simulink model "arducopter"  (R2024b)
settings: Solver=FixedStepAuto  StartTime=0.0  StopTime=simIn.param.timeEnd  FixedStep=simIn.param.dt  RelTol=1e-3
undefined symbols (not defined in the file or in its folder): DiscIntNeverNeededParam, sim, simIn
libraries: simulink x60, slident x4, vrlib x1
(part 4 of 9)

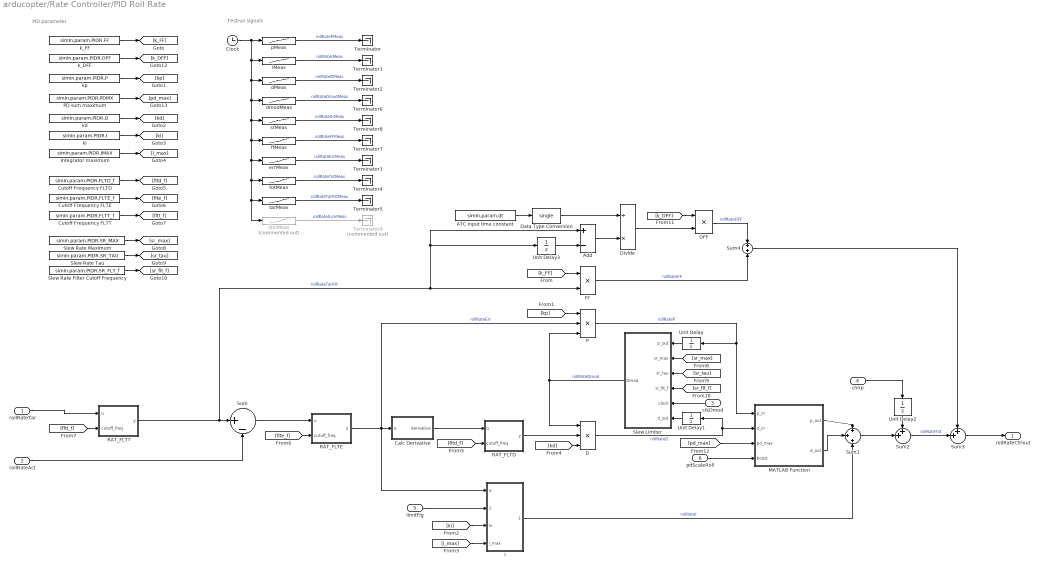
== system arducopter/Rate Controller/PID Roll Rate ==
  note: Testrun signals
  note: PID parameter
  rollRateTar : Inport
  rollRateAct : Inport  Port=2
  clkDmod : Inport  Port=3
  chirp : Inport  Port=4
  limitFlg : Inport  Port=5
  pdScaleRoll : Inport  Port=6
  ATC input time constant : Constant  Value=simIn.param.dt
  Add : Sum  Inputs=+-
  Calc Derivative : Subsystem
  Clock : Clock
  Cutoff Frequency FLTD : Constant  Value=simIn.param.PIDR.FLTD_f
  Cutoff Frequency FLTE : Constant  Value=simIn.param.PIDR.FLTE_f
  Cutoff Frequency FLTT : Constant  Value=simIn.param.PIDR.FLTT_f
  D : Product  Inputs=3
  DFF : Product
  Data Type Conversion : DataTypeConversion  OutDataTypeStr=single  SaturateOnIntegerOverflow=off  RndMeth=Floor
  Divide : Product  Inputs=/*
  FF : Product
  I : Subsystem
  Integrator maximum : Constant  Value=simIn.param.PIDR.IMAX
  MATLAB Function : MATLAB Function  TreatAsAtomicUnit=on
  P : Product  Inputs=3
  PD sum maximum : Constant  Value=simIn.param.PIDR.PDMX
  RAT_FLTD : Subsystem  TreatAsAtomicUnit=on  SystemSampleTime=simIn.param.dt
  RAT_FLTE : Subsystem  TreatAsAtomicUnit=on  SystemSampleTime=simIn.param.dt
  RAT_FLTT : Subsystem  TreatAsAtomicUnit=on  SystemSampleTime=simIn.param.dt
  Slew Limiter : Subsystem
  Slew Rate Filter Cutoff Frequency : Constant  Value=simIn.param.PIDR.SR_FLT_f
  Slew Rate Maximum : Constant  Value=simIn.param.PIDR.SR_MAX
  Slew Rate Tau : Constant  Value=simIn.param.PIDR.SR_TAU
  Sum : Sum  Inputs=|+-
  Sum1 : Sum  Inputs=+|+|+
  Sum2 : Sum  Inputs=++|
  Sum3 : Sum  Inputs=++|  OutDataTypeStr=single
  Sum4 : Sum
  Terminator{,1..8} (9 alike) : Terminator
  Terminator9 : Terminator  Commented=on
  Unit Delay : UnitDelay  InitialCondition=simIn.init.PIDR.P  SampleTime=-1  HasFrameUpgradeWarning=on
  Unit Delay1 : UnitDelay  InitialCondition=simIn.init.PIDR.D  SampleTime=-1  HasFrameUpgradeWarning=on
  Unit Delay2 : UnitDelay  SampleTime=-1  HasFrameUpgradeWarning=on
  Unit Delay3 : UnitDelay  SampleTime=-1  HasFrameUpgradeWarning=on
  dMeas : Lookup_n-D  NumberOfTableDimensions=1  BreakpointsForDimension1=simIn.signals.PIDR.Time  Table=simIn.signals.PIDR.D  InternalRulePriority=Speed  RndMeth=Simplest
  dmodMeas : Lookup_n-D  NumberOfTableDimensions=1  BreakpointsForDimension1=simIn.signals.PIDR.Time  Table=simIn.signals.PIDR.DMod  InternalRulePriority=Speed  RndMeth=Simplest
  errMeas : Lookup_n-D  NumberOfTableDimensions=1  BreakpointsForDimension1=simIn.signals.PIDR.Time  Table=simIn.signals.PIDR.Err  InternalRulePriority=Speed  RndMeth=Simplest
  ffMeas : Lookup_n-D  NumberOfTableDimensions=1  BreakpointsForDimension1=simIn.signals.PIDR.Time  Table=simIn.signals.PIDR.FF  InternalRulePriority=Speed  RndMeth=Simplest
  iMeas : Lookup_n-D  NumberOfTableDimensions=1  BreakpointsForDimension1=simIn.signals.PIDR.Time  Table=simIn.signals.PIDR.I  InternalRulePriority=Speed  RndMeth=Simplest
  ilimMeas : Lookup_n-D  Commented=on  NumberOfTableDimensions=1  BreakpointsForDimension1=simIn.signals.PIDR.Time  Table=simIn.signals.PIDR.ILimit  InternalRulePriority=Speed  RndMeth=Simplest
  k_DFF : Constant  Value=simIn.param.PIDR.DFF
  k_FF : Constant  Value=simIn.param.PIDR.FF
  kd : Constant  Value=simIn.param.PIDR.D
  ki : Constant  Value=simIn.param.PIDR.I
  kp : Constant  Value=simIn.param.PIDR.P
  pMeas : Lookup_n-D  NumberOfTableDimensions=1  BreakpointsForDimension1=simIn.signals.PIDR.Time  Table=simIn.signals.PIDR.P  InternalRulePriority=Speed  RndMeth=Simplest
  srMeas : Lookup_n-D  NumberOfTableDimensions=1  BreakpointsForDimension1=simIn.signals.PIDR.Time  Table=simIn.signals.PIDR.SRate  InternalRulePriority=Speed  RndMeth=Simplest
  tarMeas : Lookup_n-D  NumberOfTableDimensions=1  BreakpointsForDimension1=simIn.signals.PIDR.Time  Table=simIn.signals.PIDR.Tar  InternalRulePriority=Speed  RndMeth=Simplest
  totMeas : Lookup_n-D  NumberOfTableDimensions=1  BreakpointsForDimension1=simIn.signals.RATE.Time  Table=simIn.signals.RATE.ROut  InternalRulePriority=Speed  RndMeth=Simplest
  rollRateCtrlout : Outport
  wires:
  RAT_FLTD/1(y) -> D/2
  RAT_FLTE/1(y) -> P/2, Calc Derivative/1(e), I/1(e)  "rollRateErr"
  limitFlg/1 -> I/2(limit_flg)
  P/1 -> MATLAB Function/1(p_in), Unit Delay/1  "rollRateP"
  D/1 -> Unit Delay1/1, MATLAB Function/2(d_in)  "rollRateD"
  I/1(integrator) -> Sum1/3  "rollRateI"
  Sum3/1 -> rollRateCtrlout/1
  RAT_FLTT/1(y) -> Add/1, Unit Delay3/1, FF/2, Sum/1  "rollRateTarFilt"
  rollRateTar/1 -> RAT_FLTT/1(u)
  rollRateAct/1 -> Sum/2
  Sum/1 -> RAT_FLTE/1(u)
  k_FF/1 -> [k_FF]
  kp/1 -> [kp]
  kd/1 -> [kd]
  ki/1 -> [ki]
  Integrator maximum/1 -> [i_max]
  Cutoff Frequency FLTD/1 -> [fltd_f]
  Cutoff Frequency FLTE/1 -> [flte_f]
  Cutoff Frequency FLTT/1 -> [fltt_f]
  [k_FF] -> FF/1
  [kp] -> P/1
  [ki] -> I/3(ki)
  [i_max] -> I/4(i_max)
  [kd] -> D/3
  [fltd_f] -> RAT_FLTD/2(cutoff_freq)
  [flte_f] -> RAT_FLTE/2(cutoff_freq)
  [fltt_f] -> RAT_FLTT/2(cutoff_freq)
  Sum2/1 -> Sum3/2  "rollRateTot"
  pMeas/1 -> Terminator/1  "rollRatePMeas"
  iMeas/1 -> Terminator1/1  "rollRateIMeas"
  errMeas/1 -> Terminator3/1  "rollRateErrMeas"
  dMeas/1 -> Terminator2/1  "rollRateDMeas"
  tarMeas/1 -> Terminator5/1  "rollRateTarFiltMeas"
  totMeas/1 -> Terminator4/1  "rollRateTotMeas"
  Unit Delay/1 -> Slew Limiter/1(p_out)
  Unit Delay1/1 -> Slew Limiter/6(d_out)
  Slew Rate Maximum/1 -> [sr_max]
  [sr_max] -> Slew Limiter/2(sr_max)
  Slew Rate Tau/1 -> [sr_tau]
  Slew Rate Filter Cutoff Frequency/1 -> [sr_flt_f]
  [sr_tau] -> Slew Limiter/3(sr_tau)
  [sr_flt_f] -> Slew Limiter/4(sr_flt_f)
  Slew Limiter/1(Dmod) -> P/3, D/1  "rollRateDmod"
  Sum1/1 -> Sum2/2
  chirp/1 -> Unit Delay2/1
  Unit Delay2/1 -> Sum2/1
  Calc Derivative/1(derivative) -> RAT_FLTD/1(u)
  dmodMeas/1 -> Terminator6/1  "rollRateDmodMeas"
  ffMeas/1 -> Terminator7/1  "rollRateFFMeas"
  srMeas/1 -> Terminator8/1  "rollRateSrMeas"
  clkDmod/1 -> Slew Limiter/5(clock)
  ilimMeas/1 -> Terminator9/1  "rollRateILimMeas"
  Clock/1 -> ilimMeas/1, tarMeas/1, totMeas/1, errMeas/1, ffMeas/1, srMeas/1, dmodMeas/1, dMeas/1, iMeas/1, pMeas/1
  FF/1 -> Sum4/2  "rollRateFF"
  k_DFF/1 -> [k_DFF]
  Unit Delay3/1 -> Add/2
  [k_DFF] -> DFF/1
  DFF/1 -> Sum4/1  "rollRateDFF"
  Sum4/1 -> Sum3/1
  PD sum maximum/1 -> [pd_max]
  Data Type Conversion/1 -> Divide/1
  ATC input time constant/1 -> Data Type Conversion/1
  Add/1 -> Divide/2
  Divide/1 -> DFF/2
  MATLAB Function/2(d_out) -> Sum1/2
  MATLAB Function/1(p_out) -> Sum1/1
  [pd_max] -> MATLAB Function/3(pd_max)
  pdScaleRoll/1 -> MATLAB Function/4(boost)

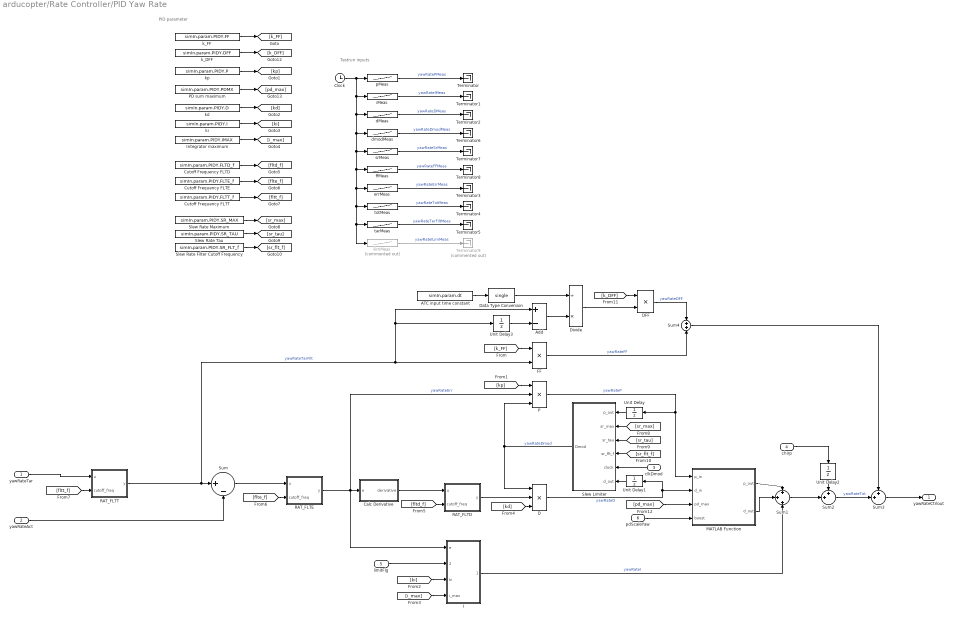
== system arducopter/Rate Controller/PID Yaw Rate ==
  note: Testrun inputs
  note: PID parameter
  yawRateTar : Inport
  yawRateAct : Inport  Port=2
  clkDmod : Inport  Port=3
  chirp : Inport  Port=4
  limitFlg : Inport  Port=5
  pdScaleYaw : Inport  Port=6
  ATC input time constant : Constant  Value=simIn.param.dt
  Add : Sum  Inputs=+-
  Calc Derivative : Subsystem
  Clock : Clock
  Cutoff Frequency FLTD : Constant  Value=simIn.param.PIDY.FLTD_f
  Cutoff Frequency FLTE : Constant  Value=simIn.param.PIDY.FLTE_f
  Cutoff Frequency FLTT : Constant  Value=simIn.param.PIDY.FLTT_f
  D : Product  Inputs=3
  DFF : Product
  Data Type Conversion : DataTypeConversion  OutDataTypeStr=single  SaturateOnIntegerOverflow=off  RndMeth=Floor
  Divide : Product  Inputs=/*
  FF : Product
  I : Subsystem
  Integrator maximum : Constant  Value=simIn.param.PIDY.IMAX
  MATLAB Function : MATLAB Function  TreatAsAtomicUnit=on
  P : Product  Inputs=3
  PD sum maximum : Constant  Value=simIn.param.PIDY.PDMX
  RAT_FLTD : Subsystem  TreatAsAtomicUnit=on  SystemSampleTime=simIn.param.dt
  RAT_FLTE : Subsystem  TreatAsAtomicUnit=on  SystemSampleTime=simIn.param.dt
  RAT_FLTT : Subsystem  TreatAsAtomicUnit=on  SystemSampleTime=simIn.param.dt
  Slew Limiter : Subsystem
  Slew Rate Filter Cutoff Frequency : Constant  Value=simIn.param.PIDY.SR_FLT_f
  Slew Rate Maximum : Constant  Value=simIn.param.PIDY.SR_MAX
  Slew Rate Tau : Constant  Value=simIn.param.PIDY.SR_TAU
  Sum : Sum  Inputs=|+-
  Sum1 : Sum  Inputs=+|+|+
  Sum2 : Sum  Inputs=++|
  Sum3 : Sum  Inputs=++|  OutDataTypeStr=single
  Sum4 : Sum
  Terminator{,1..8} (9 alike) : Terminator
  Terminator9 : Terminator  Commented=on
  Unit Delay : UnitDelay  InitialCondition=simIn.init.PIDY.P  SampleTime=-1  HasFrameUpgradeWarning=on
  Unit Delay1 : UnitDelay  InitialCondition=simIn.init.PIDY.D  SampleTime=-1  HasFrameUpgradeWarning=on
  Unit Delay2 : UnitDelay  SampleTime=-1  HasFrameUpgradeWarning=on
  Unit Delay3 : UnitDelay  SampleTime=-1  HasFrameUpgradeWarning=on
  dMeas : Lookup_n-D  NumberOfTableDimensions=1  BreakpointsForDimension1=simIn.signals.PIDY.Time  Table=simIn.signals.PIDY.D  InternalRulePriority=Speed  RndMeth=Simplest
  dmodMeas : Lookup_n-D  NumberOfTableDimensions=1  BreakpointsForDimension1=simIn.signals.PIDY.Time  Table=simIn.signals.PIDY.DMod  InternalRulePriority=Speed  RndMeth=Simplest
  errMeas : Lookup_n-D  NumberOfTableDimensions=1  BreakpointsForDimension1=simIn.signals.PIDY.Time  Table=simIn.signals.PIDY.Err  InternalRulePriority=Speed  RndMeth=Simplest
  ffMeas : Lookup_n-D  NumberOfTableDimensions=1  BreakpointsForDimension1=simIn.signals.PIDY.Time  Table=simIn.signals.PIDY.FF  InternalRulePriority=Speed  RndMeth=Simplest
  iMeas : Lookup_n-D  NumberOfTableDimensions=1  BreakpointsForDimension1=simIn.signals.PIDY.Time  Table=simIn.signals.PIDY.I  InternalRulePriority=Speed  RndMeth=Simplest
  ilimMeas : Lookup_n-D  Commented=on  NumberOfTableDimensions=1  BreakpointsForDimension1=simIn.signals.PIDY.Time  Table=simIn.signals.PIDY.ILimit  InternalRulePriority=Speed  RndMeth=Simplest
  k_DFF : Constant  Value=simIn.param.PIDY.DFF
  k_FF : Constant  Value=simIn.param.PIDY.FF
  kd : Constant  Value=simIn.param.PIDY.D
  ki : Constant  Value=simIn.param.PIDY.I
  kp : Constant  Value=simIn.param.PIDY.P
  pMeas : Lookup_n-D  NumberOfTableDimensions=1  BreakpointsForDimension1=simIn.signals.PIDY.Time  Table=simIn.signals.PIDY.P  InternalRulePriority=Speed  RndMeth=Simplest
  srMeas : Lookup_n-D  NumberOfTableDimensions=1  BreakpointsForDimension1=simIn.signals.PIDY.Time  Table=simIn.signals.PIDY.SRate  InternalRulePriority=Speed  RndMeth=Simplest
  tarMeas : Lookup_n-D  NumberOfTableDimensions=1  BreakpointsForDimension1=simIn.signals.PIDY.Time  Table=simIn.signals.PIDY.Tar  InternalRulePriority=Speed  RndMeth=Simplest
  totMeas : Lookup_n-D  NumberOfTableDimensions=1  BreakpointsForDimension1=simIn.signals.RATE.Time  Table=simIn.signals.RATE.YOut  InternalRulePriority=Speed  RndMeth=Simplest
  yawRateCtrlout : Outport
  wires:
  pMeas/1 -> Terminator/1  "yawRatePMeas"
  iMeas/1 -> Terminator1/1  "yawRateIMeas"
  dMeas/1 -> Terminator2/1  "yawRateDMeas"
  totMeas/1 -> Terminator4/1  "yawRateTotMeas"
  tarMeas/1 -> Terminator5/1  "yawRateTarFiltMeas"
  errMeas/1 -> Terminator3/1  "yawRateErrMeas"
  dmodMeas/1 -> Terminator6/1  "yawRateDmodMeas"
  srMeas/1 -> Terminator7/1  "yawRateSrMeas"
  ffMeas/1 -> Terminator8/1  "yawRateFFMeas"
  ilimMeas/1 -> Terminator9/1  "yawRateILimMeas"
  Clock/1 -> ilimMeas/1, tarMeas/1, totMeas/1, errMeas/1, ffMeas/1, srMeas/1, dmodMeas/1, dMeas/1, iMeas/1, pMeas/1
  Sum/1 -> RAT_FLTE/1(u)
  Slew Limiter/1(Dmod) -> P/3, D/1  "yawRateDmod"
  P/1 -> MATLAB Function/1(p_in), Unit Delay/1  "yawRateP"
  [fltt_f] -> RAT_FLTT/2(cutoff_freq)
  Unit Delay/1 -> Slew Limiter/1(p_out)
  FF/1 -> Sum4/2  "yawRateFF"
  DFF/1 -> Sum4/1  "yawRateDFF"
  MATLAB Function/2(d_out) -> Sum1/2
  MATLAB Function/1(p_out) -> Sum1/1
  [i_max] -> I/4(i_max)
  Calc Derivative/1(derivative) -> RAT_FLTD/1(u)
  I/1(integrator) -> Sum1/3  "yawRateI"
  Unit Delay2/1 -> Sum2/1
  [sr_tau] -> Slew Limiter/3(sr_tau)
  [flte_f] -> RAT_FLTE/2(cutoff_freq)
  [sr_flt_f] -> Slew Limiter/4(sr_flt_f)
  [pd_max] -> MATLAB Function/3(pd_max)
  Unit Delay1/1 -> Slew Limiter/6(d_out)
  [kp] -> P/1
  yawRateTar/1 -> RAT_FLTT/1(u)
  chirp/1 -> Unit Delay2/1
  D/1 -> Unit Delay1/1, MATLAB Function/2(d_in)  "yawRateD"
  RAT_FLTD/1(y) -> D/2
  [k_FF] -> FF/1
  ATC input time constant/1 -> Data Type Conversion/1
  Data Type Conversion/1 -> Divide/1
  [ki] -> I/3(ki)
  Sum3/1 -> yawRateCtrlout/1
  Add/1 -> Divide/2
  RAT_FLTE/1(y) -> P/2, Calc Derivative/1(e), I/1(e)  "yawRateErr"
  limitFlg/1 -> I/2(limit_flg)
  clkDmod/1 -> Slew Limiter/5(clock)
  [fltd_f] -> RAT_FLTD/2(cutoff_freq)
  Sum4/1 -> Sum3/1
  [k_DFF] -> DFF/1
  Sum1/1 -> Sum2/2
  [sr_max] -> Slew Limiter/2(sr_max)
  Divide/1 -> DFF/2
  [kd] -> D/3
  RAT_FLTT/1(y) -> Add/1, Unit Delay3/1, FF/2, Sum/1  "yawRateTarFilt"
  Unit Delay3/1 -> Add/2
  Sum2/1 -> Sum3/2  "yawRateTot"
  yawRateAct/1 -> Sum/2
  Integrator maximum/1 -> [i_max]
  Slew Rate Maximum/1 -> [sr_max]
  ki/1 -> [ki]
  Cutoff Frequency FLTD/1 -> [fltd_f]
  Cutoff Frequency FLTE/1 -> [flte_f]
  k_FF/1 -> [k_FF]
  Slew Rate Tau/1 -> [sr_tau]
  PD sum maximum/1 -> [pd_max]
  k_DFF/1 -> [k_DFF]
  Slew Rate Filter Cutoff Frequency/1 -> [sr_flt_f]
  kp/1 -> [kp]
  Cutoff Frequency FLTT/1 -> [fltt_f]
  kd/1 -> [kd]
  pdScaleYaw/1 -> MATLAB Function/4(boost)

== system arducopter/Throttle/Input Handler ==
  note: Input Handler
      | Determines source of the inputs to the subsystem, which can
      | be either the real flight data or simulated data.
  inMeas : Inport
  inSim : Inport  Port=2
  thrMan : Inport  Port=3
  Bus Creator : BusCreator  Inputs=9
  Bus Selector : BusSelector  OutputSignals=throttle.thrIn
  Bus Selector1 : BusSelector  OutputSignals=CTUN.thrInMeas,CTUN.angBst,BAT.batRestVoltEst,BAT.batCurr,BAT.batRes,BAT.batVolt,BARO.baroAlt,BARO.baroAirPress,BARO.baroGndTemp
  Switch : Switch  Criteria=u2 > Threshold  SaturateOnIntegerOverflow=off  InputSameDT=off
  data_in : Outport
  wires:
  inSim/1 -> Bus Selector/1
  inMeas/1 -> Bus Selector1/1
  thrMan/1 -> Switch/2
  Bus Selector/1 -> Switch/3  "<thrIn>"
  Bus Selector1/1 -> Switch/1  "<thrInMeas>"
  Bus Selector1/9 -> Bus Creator/9  "<baroGndTemp>"
  Bus Selector1/8 -> Bus Creator/8  "<baroAirPress>"
  Bus Selector1/7 -> Bus Creator/7  "<baroAlt>"
  Bus Selector1/6 -> Bus Creator/6  "<batVolt>"
  Bus Selector1/5 -> Bus Creator/5  "<batRes>"
  Bus Selector1/4 -> Bus Creator/4  "<batCurr>"
  Bus Selector1/3 -> Bus Creator/3  "<batRestVoltEst>"
  Bus Selector1/2 -> Bus Creator/2  "<angBst>"
  Switch/1 -> Bus Creator/1  "thrTar"
  Bus Creator/1 -> data_in/1

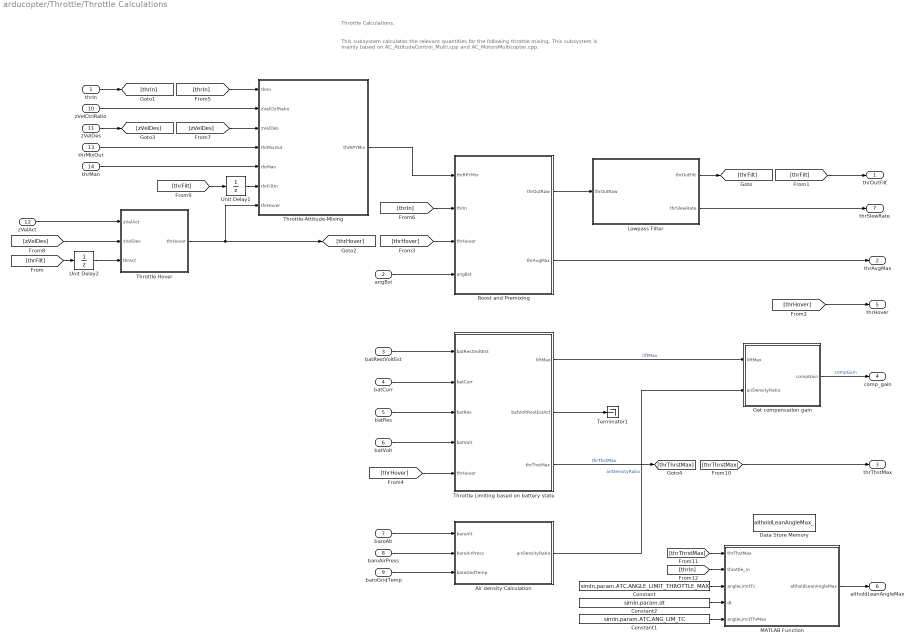
== system arducopter/Throttle/Throttle Calculations ==
  note: Throttle Calculations.
  note: This subsystem calculates the relevant quantities for the following throttle mixing.
      | This subsystem is mainly based on AC_AttitudeControl_Multi.cpp and AC_MotorsMulticopter.cpp.
  thrIn : Inport
  angBst : Inport  Port=2
  batRestVoltEst : Inport  Port=3
  batCurr : Inport  Port=4
  batRes : Inport  Port=5
  batVolt : Inport  Port=6
  baroAlt : Inport  Port=7
  baroAirPress : Inport  Port=8
  baroGndTemp : Inport  Port=9
  zVelCtrlRatio : Inport  Port=10
  zVelDes : Inport  Port=11
  zVelAct : Inport  Port=12
  thrMixOut : Inport  Port=13
  thrMan : Inport  Port=14
  Air density Calculation : Subsystem
  Boost and Premixing : Subsystem  TreatAsAtomicUnit=on  SystemSampleTime=simIn.param.dt
  Constant : Constant  Value=simIn.param.ATC.ANGLE_LIMIT_THROTTLE_MAX
  Constant1 : Constant  Value=simIn.param.ATC.ANG_LIM_TC
  Constant2 : Constant  Value=simIn.param.dt
  Data Store Memory : DataStoreMemory  DataStoreName=altholdLeanAngleMax_  ReadBeforeWriteMsg=warning  WriteAfterWriteMsg=warning  WriteAfterReadMsg=warning  InitialValue=single(0)  ShowAdditionalParam=off  OutDataTypeStr=single
  Get compensation gain : MATLAB Function  TreatAsAtomicUnit=on
  Lowpass Filter : Subsystem
  MATLAB Function : MATLAB Function  TreatAsAtomicUnit=on
  Terminator1 : Terminator
  Throttle Hover : Subsystem  TreatAsAtomicUnit=on  SystemSampleTime=0.1
  Throttle Limiting based on battery state : Subsystem
  Throttle-Attitude-Mixing : Subsystem
  Unit Delay1 : UnitDelay  InitialCondition=simIn.init.CTUN.ThrOut  SampleTime=-1  HasFrameUpgradeWarning=on
  Unit Delay2 : UnitDelay  InitialCondition=simIn.init.CTUN.ThrOut  SampleTime=-1  HasFrameUpgradeWarning=on
  thrOutFilt : Outport
  thrAvgMax : Outport  Port=2
  thrThstMax : Outport  Port=3
  comp_gain : Outport  Port=4
  thrHover : Outport  Port=5
  altholdLeanAngleMax : Outport  Port=6
  thrSlewRate : Outport  Port=7
  wires:
  Throttle Hover/1(thrHover) -> [thrHover], Throttle-Attitude-Mixing/7(thrHover)
  Get compensation gain/1(compGain) -> comp_gain/1  "compGain"
  Throttle Limiting based on battery state/1(liftMax) -> Get compensation gain/1(liftMax)  "liftMax"
  [thrFilt] -> Unit Delay2/1
  Throttle Limiting based on battery state/2(batVoltRestEstAct) -> Terminator1/1
  [thrHover] -> Throttle Limiting based on battery state/5(thrHover)
  Unit Delay2/1 -> Throttle Hover/3(thrAct)
  Throttle Limiting based on battery state/3(thrThstMax) -> [thrThrstMax]  "thrThstMax"
  [thrFilt] -> thrOutFilt/1
  Lowpass Filter/1(thrOutFilt) -> [thrFilt]
  angBst/1 -> Boost and Premixing/4(angBst)
  [thrHover] -> Boost and Premixing/3(thrHover)
  Boost and Premixing/2(thrAvgMax) -> thrAvgMax/1
  batRestVoltEst/1 -> Throttle Limiting based on battery state/1(batRestVoltEst)
  batCurr/1 -> Throttle Limiting based on battery state/2(batCurr)
  batRes/1 -> Throttle Limiting based on battery state/3(batRes)
  batVolt/1 -> Throttle Limiting based on battery state/4(batVolt)
  baroAlt/1 -> Air density Calculation/1(baroAlt)
  baroAirPress/1 -> Air density Calculation/2(baroAirPress)
  baroGndTemp/1 -> Air density Calculation/3(baroGndTemp)
  Boost and Premixing/1(thrOutRaw) -> Lowpass Filter/1(thrOutRaw)
  [thrHover] -> thrHover/1
  [thrIn] -> Boost and Premixing/2(thrIn)
  thrIn/1 -> [thrIn]
  zVelCtrlRatio/1 -> Throttle-Attitude-Mixing/2(zVelCtrlRatio)
  thrMan/1 -> Throttle-Attitude-Mixing/5(thrMan)
  Throttle-Attitude-Mixing/1(thrRPYMix) -> Boost and Premixing/1(thrRPYMix)
  [thrIn] -> Throttle-Attitude-Mixing/1(thrIn)
  zVelDes/1 -> [zVelDes]
  [zVelDes] -> Throttle-Attitude-Mixing/3(zVelDes)
  [zVelDes] -> Throttle Hover/2(zVelDes)
  zVelAct/1 -> Throttle Hover/1(zVelAct)
  Air density Calculation/1(airDensityRatio) -> Get compensation gain/2(airDensityRatio)  "airDensityRatio"
  thrMixOut/1 -> Throttle-Attitude-Mixing/4(thrMixOut)
  [thrFilt] -> Unit Delay1/1
  Unit Delay1/1 -> Throttle-Attitude-Mixing/6(thrFiltIn)
  [thrThrstMax] -> thrThstMax/1
  [thrThrstMax] -> MATLAB Function/1(thrThstMax)
  [thrIn] -> MATLAB Function/2(throttle_in)
  Constant/1 -> MATLAB Function/3(angleLimitTc)
  Constant1/1 -> MATLAB Function/5(angleLimitThrMax)
  Constant2/1 -> MATLAB Function/4(dt)
  MATLAB Function/1(altholdLeanAngleMax) -> altholdLeanAngleMax/1
  Lowpass Filter/2(thrSlewRate) -> thrSlewRate/1

== system arducopter/Attitude Controller/input_euler_angle_roll_pitch_euler_rate_yaw()/Add feedforward to angVelBody ==
  note: Thrust error angle above which yaw corrections are limited
  angVelBodyFeedforward : Inport
  angVelBodyIn : Inport  Port=2
  thurstErrorAngle : Inport  Port=3
  yawRateAct : Inport  Port=4
  Constant : Constant  Value=simIn.param.ATC.THRUST_ERROR_ANGLE
  MATLAB Function : MATLAB Function  TreatAsAtomicUnit=on
  angVelBody : Outport
  feedforwardScaler : Outport  Port=2
  wires:
  angVelBodyFeedforward/1 -> MATLAB Function/1(angVelBodyFeedforward)
  angVelBodyIn/1 -> MATLAB Function/2(angVelBodyIn)
  thurstErrorAngle/1 -> MATLAB Function/3(thrustErrorAngle)
  yawRateAct/1 -> MATLAB Function/4(yawRateAct)
  MATLAB Function/1(angVelBodyNew) -> angVelBody/1
  Constant/1 -> MATLAB Function/5(maxThrustErrorAngle4YawCorr)
  MATLAB Function/2(feedforwardScaler) -> feedforwardScaler/1

== system arducopter/Attitude Controller/input_euler_angle_roll_pitch_euler_rate_yaw()/Feedforward disabled ==
  note: QuaternionT<T>::from_euler()
      | Computes the quaternion from the given euler angles
  note: This subsystem represents to part of input_euler_angle_roll_pitch_euler_rate_yaw() that is executed, when the feedforward is disabled ( ATC_RATE_FF_ENAB = 0 )
  eulerAngleTar : Inport
  eulerInputDes : Inport  Port=2
  Constant : Constant  Value=0  OutDataTypeStr=single
  Constant1 : Constant  Value=0  OutDataTypeStr=single
  Demux : Demux  Outputs=3
  Gain : Gain  Gain=simIn.param.dt
  MATLAB Function : MATLAB Function  TreatAsAtomicUnit=on
  Selector : Selector  InputPortWidth=3  IndexOptions=Index vector (dialog)  Indices=[3]  OutputSizes=1
  Sum : Sum  Inputs=|++
  eulerRateTar : Outport
  angVelTar : Outport  Port=2
  attitudeTarget : Outport  Port=3
  wires:
  MATLAB Function/1(q) -> attitudeTarget/1  "attitudeTarget"
  Demux/1 -> MATLAB Function/1(roll)
  Demux/2 -> MATLAB Function/2(pitch)
  eulerInputDes/1 -> Demux/1
  Demux/3 -> Gain/1
  Gain/1 -> Sum/1
  Sum/1 -> MATLAB Function/3(yaw)
  eulerAngleTar/1 -> Selector/1
  Constant/1 -> eulerRateTar/1
  Constant1/1 -> angVelTar/1
  Selector/1 -> Sum/2

== system arducopter/Attitude Controller/input_euler_angle_roll_pitch_euler_rate_yaw()/Feedforward enabled ==
  note: direkt _attitude_target statt euler_angle_target
  note: euler_rate_to_ang_vel()
      | Converts the target euler rates into a target frame angular velocity vector for feedforward
  note: euler_accel_limit()
      | Translation of acceleration limits eulerAccelMax to the body frame
  note: This subsystem represents to part of input_euler_angle_roll_pitch_euler_rate_yaw() that is executed, when the feedforward is enabled (ATC_RATE_FF_ENAB = 1)
  note: Maximum angular accelerations in earth frame
  note: Input shaping
      | Computes target euler rates based on the error between latest angle target and the desired angle by the pilot, thereby considering acceleration limits.
  note: ang_vel_limit()
      | Ensures that angular velocites do not go over configured rate limits
  note: ang_vel_to_euler_rate()
      | Converts the target body-frame angular velocites into target euler rates
  eulerRateTarIn : Inport
  eulerAngleTar : Inport  Port=2
  eulerInputDes : Inport  Port=3
  Constant : Constant  Value=simIn.param.ATC.ACCEL_R_MAX
  Constant1 : Constant  Value=simIn.param.ATC.ACCEL_P_MAX
  Constant2 : Constant  Value=simIn.param.ATC.ACCEL_Y_MAX
  Constant3 : Constant  Value=simIn.param.ATC.RATE_R_MAX
  Constant4 : Constant  Value=simIn.param.ATC.RATE_P_MAX
  Constant5 : Constant  Value=simIn.param.ATC.RATE_Y_MAX
  Gain : Gain  Gain=pi/180
  Gain1 : Gain  Gain=pi/180
  Gain2 : Gain  Gain=pi/180
  MATLAB Function : MATLAB Function  TreatAsAtomicUnit=on
  MATLAB Function1 : MATLAB Function  TreatAsAtomicUnit=on
  MATLAB Function2 : MATLAB Function  TreatAsAtomicUnit=on
  MATLAB Function3 : MATLAB Function  TreatAsAtomicUnit=on
  Mux : Mux  Inputs=3
  cdeg/ss to rad/ss : Gain  Gain=0.01*pi/180
  input shaping : Subsystem
  eulerRateTarOut : Outport
  angVelTar : Outport  Port=2
  wires:
  [eulerAngleTar] -> MATLAB Function/1(eulerAngleTar), MATLAB Function1/1(eulerAngle), input shaping/1(eulerAngleTar)
  Constant/1 -> Mux/1
  Mux/1 -> cdeg/ss to rad/ss/1
  Constant1/1 -> Mux/2
  Constant2/1 -> Mux/3
  MATLAB Function/1(eulerAccelMaxBF) -> input shaping/4(eulerAccelMax)
  eulerInputDes/1 -> input shaping/2(eulerInputDes)
  eulerRateTarIn/1 -> input shaping/3(eulerRateTarIn)
  input shaping/1(eulerRateTar) -> MATLAB Function1/2(eulerRate)  "eulerRateTar"
  MATLAB Function1/1(angVelTar) -> MATLAB Function2/1(angVelTar)  "angVelTar"
  Gain/1 -> MATLAB Function2/2(angVelRollMax)
  Constant3/1 -> Gain/1
  Constant4/1 -> Gain1/1
  Gain1/1 -> MATLAB Function2/3(angVelPitchMax)
  Gain2/1 -> MATLAB Function2/4(angVelYawMax)
  Constant5/1 -> Gain2/1
  eulerAngleTar/1 -> [eulerAngleTar]  "eulerAngleTar"
  [eulerAngleTar] -> MATLAB Function3/2(eulerAngle)
  MATLAB Function3/1(eulerRate) -> eulerRateTarOut/1
  MATLAB Function2/1(angVelTarLimited) -> [angVelTar]
  [angVelTar] -> MATLAB Function3/1(angVelBf)
  [angVelTar] -> angVelTar/1
  cdeg/ss to rad/ss/1 -> MATLAB Function/2(eulerAccelMaxEF)

== system arducopter/Attitude Controller/input_euler_angle_roll_pitch_euler_rate_yaw()/Update attitudeTarget ==
  note: Normalize attitudeTarget
  note: Use angVelTar to rotate attitudeTarget
  note: Use rotated attitudeTarget, if FF is enabled.
      | Otherwise, use unchanged attitudeTarget
  attitudeTarget : Inport
  angVelTar : Inport  Port=2
  ffEnabled : Inport  Port=3
  MATLAB Function : MATLAB Function  TreatAsAtomicUnit=on
  Rotate target attitude : Subsystem
  Switch : Switch  Criteria=u2 > Threshold  SaturateOnIntegerOverflow=off  InputSameDT=off
  attitudeTargetUpdate : Outport
  wires:
  MATLAB Function/1(qNorm) -> attitudeTargetUpdate/1
  Switch/1 -> MATLAB Function/1(q)
  ffEnabled/1 -> Switch/2
  attitudeTarget/1 -> Switch/3, Rotate target attitude/1(attitudeTarget)
  angVelTar/1 -> Rotate target attitude/2(angVelTar)
  Rotate target attitude/1(attitudeTargetRot) -> Switch/1

== system arducopter/Attitude Controller/input_euler_angle_roll_pitch_euler_rate_yaw()/reset yaw targets ==
  note: Anmerkung:
      | euler_rate_to_ang_vel(_euler_angle_target, _euler_rate_target, _ang_vel_target);
      | zu
      | euler_rate_to_ang_vel(_attitude_target, _euler_rate_target, _ang_vel_target);
      |
      | wird hier generell nicht hier berücksichtigt
      | Änderung bewirkt, dass der aktualisierte Quaternion als Input genommen wird und nicht die "nicht aktualisierten" Eulerwinkel. Würde sich auf Winkelgeschwindigkeiten auswirken
  note: "ahrs.yaw - euler_angle_target.z"
  note: This subsystem resets the yaw target angle and rate, if the throttle is zero, meaning that the copter is landed. The respective function is AC_AttitudeControl::reset_yaw_target_and_rate() , which is called in ModeStabilize::run() when the copter is armed, but throttle is still zero.
  eulerRateTarIn : Inport
  attitudeTargetIn : Inport  Port=2
  eulerAngleAct : Inport  Port=3
  throttle : Inport  Port=4
  Demux : Demux  Outputs=3
  Demux1 : Demux  Outputs=3
  MATLAB Function1 : MATLAB Function  TreatAsAtomicUnit=on
  MATLAB Function5 : MATLAB Function  TreatAsAtomicUnit=on
  MATLAB Function9 : MATLAB Function  TreatAsAtomicUnit=on
  Mux : Mux  Inputs=3
  Mux1 : Mux  Inputs=3
  Subtract : Sum  Inputs=-+
  Switch : Switch  Criteria=u2 > Threshold  SaturateOnIntegerOverflow=off  InputSameDT=off
  Switch1 : Switch  Criteria=u2 > Threshold  SaturateOnIntegerOverflow=off  InputSameDT=off
  Terminator{,1..4} (5 alike) : Terminator
  Zero : Constant  Value=0  OutDataTypeStr=single
  Zero1 : Constant  Value=0  OutDataTypeStr=single
  Zero2 : Constant  Value=0  OutDataTypeStr=single
  eulerRateTar : Outport
  attitudeTarget : Outport  Port=2
  wires:
  Switch1/1 -> attitudeTarget/1
  Switch/1 -> eulerRateTar/1
  throttle/1 -> Switch1/2, Switch/2
  eulerRateTarIn/1 -> Demux1/1, Switch/1
  eulerAngleAct/1 -> Demux/1
  MATLAB Function9/1(qRes) -> Switch1/3
  attitudeTargetIn/1 -> Switch1/1, MATLAB Function9/2(q2), MATLAB Function1/1(q)
  MATLAB Function1/3(yaw) -> Subtract/1  "yawAngleTar"
  MATLAB Function1/1(roll) -> Terminator/1
  MATLAB Function1/2(pitch) -> Terminator1/1
  Demux/1 -> Terminator2/1
  Demux/2 -> Terminator3/1
  Demux/3 -> Subtract/2
  Subtract/1 -> Mux/3
  MATLAB Function5/1(q) -> MATLAB Function9/1(q1)  "attitudeTargetUpdate"
  Mux/1 -> MATLAB Function5/1(vec)
  Zero/1 -> Mux/1
  Zero1/1 -> Mux/2
  Mux1/1 -> Switch/3
  Demux1/1 -> Mux1/1
  Demux1/2 -> Mux1/2
  Demux1/3 -> Terminator4/1
  Zero2/1 -> Mux1/3

== system arducopter/Attitude Controller/input_euler_angle_roll_pitch_euler_rate_yaw()/thrust_heading_rotation_angles() ==
  note: Limit yaw error based in maximum acceleration
  note: AC_AttitudeControl::thrust_vector_rotation_angles()
      | Calculation of thrust_angle, thrust_error_angle, attitude_error and thrust_vector_correction
  note: This subsystem contains all the calculations contained in the function AC_AttitudeControl::thrust_heading_rotation_angles() that is called in AC_AttitudeControl::attitude_controller_run_quat()
  attitudeTargetIn : Inport
  attitudeBodyAct : Inport  Port=2
  Yaw error limitation : Subsystem
  thrust_vector_rotation_angles() : Subsystem
  attitudeTarget : Outport
  attitudeError : Outport  Port=2
  thrustErrorAngle : Outport  Port=3
  thrustAngle : Outport  Port=4
  wires:
  attitudeTargetIn/1 -> [attitudeTarget]  "attTar"
  [attitudeBody] -> thrust_vector_rotation_angles()/2(attitudeBodyAct)
  thrust_vector_rotation_angles()/1(attitudeError) -> Yaw error limitation/1(attitudeErrorIn)
  thrust_vector_rotation_angles()/3(thrustErrAngle) -> thrustErrorAngle/1
  thrust_vector_rotation_angles()/2(thrustVecCorrection) -> Yaw error limitation/3(thrustVecCorrection)
  thrust_vector_rotation_angles()/4(thrustAngle) -> thrustAngle/1
  attitudeBodyAct/1 -> [attitudeBody]  "attBody"
  [attitudeBody] -> Yaw error limitation/4(attitudeBody)
  Yaw error limitation/1(attitudeTarget) -> attitudeTarget/1
  Yaw error limitation/2(attitudeError) -> attitudeError/1
  [attitudeTarget] -> thrust_vector_rotation_angles()/1(attitudeTarget)
  [attitudeTarget] -> Yaw error limitation/2(attitudeTargetIn)

== system arducopter/Attitude Controller/input_euler_angle_roll_pitch_euler_rate_yaw()/update_ang_vel_target_from_att_error() ==
  note: The subsystems either use the square root controller or an easy proportional relation (kp*err) to calculate the target angular velocity
  note: AC_AttitudeControl::update_ang_vel_target_from_att_error()
      | Compute the angular velocity corrections in the body frame from the attitude error.
  attitudeError : Inport
  anglePScale : Inport  Port=2
  Calc angular velocity target pitch : Subsystem
  Calc angular velocity target roll : Subsystem
  Calc angular velocity target yaw : Subsystem
  Mux : Mux  Inputs=3
  Selector : Selector  InputPortWidth=3  IndexOptions=Index vector (dialog)  Indices=[1]  OutputSizes=1
  Selector1 : Selector  InputPortWidth=3  IndexOptions=Index vector (dialog)  Indices=[2]  OutputSizes=1
  Selector2 : Selector  InputPortWidth=3  IndexOptions=Index vector (dialog)  Indices=[3]  OutputSizes=1
  Selector3 : Selector  InputPortWidth=3  IndexOptions=Index vector (dialog)  Indices=[2]  OutputSizes=1
  Selector4 : Selector  InputPortWidth=3  IndexOptions=Index vector (dialog)  Indices=[1]  OutputSizes=1
  angVelBody : Outport
  wires:
  attitudeError/1 -> Selector2/1, Selector/1, Selector1/1
  Mux/1 -> angVelBody/1
  Selector/1 -> Calc angular velocity target roll/1(attitudeErrorRoll)
  Calc angular velocity target roll/1(angVelRoll) -> Mux/1
  Calc angular velocity target yaw/1(angVelYaw) -> Mux/3
  Calc angular velocity target pitch/1(angVelPitch) -> Mux/2
  Selector1/1 -> Calc angular velocity target pitch/1(attitudeErrorPitch)
  Selector2/1 -> Calc angular velocity target yaw/1(attitudeErrorYaw)
  anglePScale/1 -> Selector3/1, Selector4/1
  Selector4/1 -> Calc angular velocity target roll/2(anglePScale)
  Selector3/1 -> Calc angular velocity target pitch/2(anglePScale)

== system arducopter/Position Controller/P Position z/Scale Factor Z ==
  note: AP_AHRS::getControlScaleZ()
      | This subsystem calculates a scaling factor for the target of vertical motion quantities based on the EKF type that is being used.
      | Taken from AP_AHRS::getControlScaleZ() in AP_AHRS.cpp. Called in AC_PosControl::update_z_controller().
      | Flying with only DCM lower the gain of the controllers by 4x to cope with high lag.
  ekfType : Inport
  EKF used : Constant  OutDataTypeStr=single
  No EKF : Constant  Value=0.25  OutDataTypeStr=single
  Switch : Switch  Criteria=u2 > Threshold  SaturateOnIntegerOverflow=off  InputSameDT=off
  scale_z : Outport
  wires:
  ekfType/1 -> Switch/2
  EKF used/1 -> Switch/1
  No EKF/1 -> Switch/3
  Switch/1 -> scale_z/1

== system arducopter/Position Controller/P Position z/Set vertical speed & acceleration limit ==
  note: Calculation of vertical speed and acceleration limits
      | This subsystem corresponds to the function set_correction_speed_accel_z() , in AC_PosControl.cpp,
      | which is called in the ModeLoiter::init() function of mode_loiter.cpp.
      | The intention of this function is to calculate z position error limits, which corresponds to the vertical speed
      | and acceleration limits given by parameters, so that the speed and acceleration limits are still kept after
      | the square root controller was executed without explicitly enforce the limits to the quantities.
  outMin : Inport
  outMax : Inport  Port=2
  DoutMax : Inport  Port=3
  D2OutMax : Inport  Port=4
  kp : Inport  Port=5
  Abs : Abs  SaturateOnIntegerOverflow=off
  Gain : Gain  Gain=-1
  Inverse Square Root Controller : Subsystem  TreatAsAtomicUnit=on
  Set error limits : MATLAB Function  TreatAsAtomicUnit=on
  errMin : Outport
  errMax : Outport  Port=2
  D1max : Outport  Port=3
  wires:
  Abs/1 -> Gain/1
  Gain/1 -> Set error limits/1(outMin)
  outMax/1 -> Set error limits/2(outMax)
  outMin/1 -> Abs/1
  DoutMax/1 -> Set error limits/3(DoutMax)
  Set error limits/1(errMin) -> errMin/1
  Set error limits/3(D1max) -> D1max/1
  Set error limits/2(errMax) -> errMax/1
  D2OutMax/1 -> Set error limits/4(D2OutMax)
  kp/1 -> Set error limits/5(kp)

== system arducopter/Position Controller/PID Acceleration z/Calc Derivative ==
  e : Inport
  ATC input time constant : Constant  Value=simIn.param.dt
  Divide : Product  Inputs=*/
  Sum : Sum  Inputs=|+-
  Unit Delay : UnitDelay  SampleTime=-1  HasFrameUpgradeWarning=on
  derivative : Outport
  wires:
  e/1 -> Sum/1, Unit Delay/1
  Unit Delay/1 -> Sum/2
  Sum/1 -> Divide/1
  ATC input time constant/1 -> Divide/2
  Divide/1 -> derivative/1

== system arducopter/Position Controller/PID Acceleration z/I ==
  note: Integrator, see AC_PID.cpp, line 230
      | Initialization: set_integrator() in AC_PosControl::init_z_controller()
  e : Inport
  limitFlg : Inport  Port=2
  ki : Inport  Port=3
  i_max : Inport  Port=4
  Constant1 : Constant  Value=simIn.param.dt
  Data Type Conversion1 : DataTypeConversion  OutDataTypeStr=single  SaturateOnIntegerOverflow=off  RndMeth=Floor
  IC1 : InitialCondition  Value=simIn.init.PIDA.I
  Integrator : MATLAB Function  TreatAsAtomicUnit=on
  Unit Delay1 : UnitDelay  InitialCondition=simIn.init.PIDA.I  SampleTime=-1  HasFrameUpgradeWarning=on
  integrator : Outport
  wires:
  e/1 -> Integrator/1(error)
  Integrator/1(integrator_out) -> IC1/1
  [integrator_out] -> integrator/1
  Constant1/1 -> Data Type Conversion1/1
  limitFlg/1 -> Integrator/3(limit_flg)
  [integrator_out] -> Unit Delay1/1
  IC1/1 -> [integrator_out]
  Unit Delay1/1 -> Integrator/2(integrator)
  ki/1 -> Integrator/4(ki)
  i_max/1 -> Integrator/5(i_max)
  Data Type Conversion1/1 -> Integrator/6(dt)

== system arducopter/Position Controller/PID Acceleration z/RAT_FLTD ==
  note: Digital Filter:
      | $y_n = (1 - \alpha)y_{n-1} + x \cdot \alpha$
  note: See AC_PID.cpp, line 144.
  note: See AP_Math.cpp, calc_lowpass_alpha_dt()
  note: Alpha Calculation:
      | $\alpha = \frac{\mathrm{d}t}{\mathrm{d}t + 2 \pi f_{\mathrm{Cutoff}}$
  u : Inport
  cutoff_freq : Inport  Port=2
  ATC input time constant1 : Constant  Value=simIn.param.dt
  Add1 : Sum
  Calculate Alpha1 : Product  Inputs=*/
  Compare To Zero2 : simulink/Logic and Bit Operations/Compare To Zero  relop=<=  OutDataTypeStr=boolean
  Compare To Zero3 : simulink/Logic and Bit Operations/Compare To Zero  relop=<=  OutDataTypeStr=boolean
  Compare To Zero4 : simulink/Logic and Bit Operations/Compare To Zero  relop=~=  OutDataTypeStr=boolean
  Constant1 : Constant  OutDataTypeStr=single
  Constant2 : Constant  OutDataTypeStr=single
  Constant5 : Constant  OutDataTypeStr=single
  Data Type Conversion1 : DataTypeConversion  OutDataTypeStr=single  SaturateOnIntegerOverflow=off  RndMeth=Floor
  Divide1 : Product  Inputs=*/
  Gain1 : Gain  Gain=2*pi
  IC : InitialCondition  Value=simIn.init.PIDA.DerFilt
  Logical Operator1 : Logic  Operator=OR  AllPortsSameDT=off  OutDataTypeStr=boolean
  Product : Product
  Product1 : Product
  Product2 : Product
  Subtract1 : Sum  Inputs=+-
  Sum : Sum  Inputs=++|  OutDataTypeStr=single
  Switch1 : Switch  Criteria=u2 > Threshold  SaturateOnIntegerOverflow=off  InputSameDT=off
  Unit Delay : UnitDelay  SampleTime=-1  HasFrameUpgradeWarning=on
  y : Outport
  wires:
  Product1/1 -> Sum/2
  Unit Delay/1 -> Product1/2
  Subtract1/1 -> Product1/1
  [alpha] -> Subtract1/2
  Constant2/1 -> Subtract1/1
  [alpha] -> Product/1
  u/1 -> Product/2
  Product/1 -> Sum/1
  Sum/1 -> IC/1
  IC/1 -> Unit Delay/1, y/1
  [dt] -> Compare To Zero2/1
  Constant1/1 -> Divide1/1
  Divide1/1 -> Add1/2
  Product2/1 -> Switch1/1
  Add1/1 -> Calculate Alpha1/2
  Gain1/1 -> Divide1/2
  Compare To Zero3/1 -> Logical Operator1/2
  [dt] -> Compare To Zero4/1
  Data Type Conversion1/1 -> [dt]
  ATC input time constant1/1 -> Data Type Conversion1/1
  [cutoff_freq] -> Gain1/1
  Switch1/1 -> [alpha]
  [dt] -> Calculate Alpha1/1, Add1/1
  Compare To Zero4/1 -> Product2/1
  cutoff_freq/1 -> [cutoff_freq]
  Compare To Zero2/1 -> Logical Operator1/1
  [cutoff_freq] -> Compare To Zero3/1
  Calculate Alpha1/1 -> Switch1/3
  Logical Operator1/1 -> Switch1/2
  Constant5/1 -> Product2/2

== system arducopter/Position Controller/PID Acceleration z/RAT_FLTE ==
  note: Digital Filter:
      | $y_n = (1 - \alpha)y_{n-1} + x \cdot \alpha$
  note: See AC_PID.cpp, line 144.
  note: See AP_Math.cpp, calc_lowpass_alpha_dt()
  note: Alpha Calculation:
      | $\alpha = \frac{\mathrm{d}t}{\mathrm{d}t + 2 \pi f_{\mathrm{Cutoff}}$
  u : Inport
  cutoff_freq : Inport  Port=2
  ATC input time constant1 : Constant  Value=simIn.param.dt
  Add1 : Sum
  Calculate Alpha1 : Product  Inputs=*/
  Compare To Zero2 : simulink/Logic and Bit Operations/Compare To Zero  relop=<=  OutDataTypeStr=boolean
  Compare To Zero3 : simulink/Logic and Bit Operations/Compare To Zero  relop=<=  OutDataTypeStr=boolean
  Compare To Zero4 : simulink/Logic and Bit Operations/Compare To Zero  relop=~=  OutDataTypeStr=boolean
  Constant1 : Constant  OutDataTypeStr=single
  Constant2 : Constant  OutDataTypeStr=single
  Constant5 : Constant  OutDataTypeStr=single
  Data Type Conversion1 : DataTypeConversion  OutDataTypeStr=single  SaturateOnIntegerOverflow=off  RndMeth=Floor
  Divide1 : Product  Inputs=*/
  Gain1 : Gain  Gain=2*pi
  IC : InitialCondition  Value=simIn.init.PIDA.ErrFilt
  Logical Operator1 : Logic  Operator=OR  AllPortsSameDT=off  OutDataTypeStr=boolean
  Product : Product
  Product1 : Product
  Product2 : Product
  Subtract1 : Sum  Inputs=+-
  Sum : Sum  Inputs=++|  OutDataTypeStr=single
  Switch1 : Switch  Criteria=u2 > Threshold  SaturateOnIntegerOverflow=off  InputSameDT=off
  Unit Delay : UnitDelay  SampleTime=-1  HasFrameUpgradeWarning=on
  y : Outport
  wires:
  Product1/1 -> Sum/2
  Unit Delay/1 -> Product1/2
  Subtract1/1 -> Product1/1
  [alpha] -> Subtract1/2
  Constant2/1 -> Subtract1/1
  [alpha] -> Product/1
  u/1 -> Product/2
  Product/1 -> Sum/1
  Sum/1 -> IC/1
  IC/1 -> Unit Delay/1, y/1
  [dt] -> Compare To Zero2/1
  Constant1/1 -> Divide1/1
  Divide1/1 -> Add1/2
  Product2/1 -> Switch1/1
  Add1/1 -> Calculate Alpha1/2
  Gain1/1 -> Divide1/2
  Compare To Zero3/1 -> Logical Operator1/2
  [dt] -> Compare To Zero4/1
  Data Type Conversion1/1 -> [dt]
  ATC input time constant1/1 -> Data Type Conversion1/1
  [cutoff_freq] -> Gain1/1
  Switch1/1 -> [alpha]
  [dt] -> Calculate Alpha1/1, Add1/1
  Compare To Zero4/1 -> Product2/1
  cutoff_freq/1 -> [cutoff_freq]
  Compare To Zero2/1 -> Logical Operator1/1
  [cutoff_freq] -> Compare To Zero3/1
  Calculate Alpha1/1 -> Switch1/3
  Logical Operator1/1 -> Switch1/2
  Constant5/1 -> Product2/2

== system arducopter/Position Controller/PID Acceleration z/RAT_FLTT ==
  note: See AC_PID.cpp, line 144.
  note: Digital Filter:
      | $y_n = (1 - \alpha)y_{n-1} + x \cdot \alpha$
  note: See AP_Math.cpp, calc_lowpass_alpha_dt()
  note: Alpha Calculation:
      | $\alpha = \frac{\mathrm{d}t}{\mathrm{d}t + 2 \pi f_{\mathrm{Cutoff}}$
  u : Inport
  cutoff_freq : Inport  Port=2
  ATC input time constant1 : Constant  Value=simIn.param.dt
  Add1 : Sum
  Calculate Alpha1 : Product  Inputs=*/
  Compare To Zero2 : simulink/Logic and Bit Operations/Compare To Zero  relop=<=  OutDataTypeStr=boolean
  Compare To Zero3 : simulink/Logic and Bit Operations/Compare To Zero  relop=<=  OutDataTypeStr=boolean
  Compare To Zero4 : simulink/Logic and Bit Operations/Compare To Zero  relop=~=  OutDataTypeStr=boolean
  Constant1 : Constant  OutDataTypeStr=single
  Constant2 : Constant  OutDataTypeStr=single
  Constant5 : Constant  OutDataTypeStr=single
  Data Type Conversion1 : DataTypeConversion  OutDataTypeStr=single  SaturateOnIntegerOverflow=off  RndMeth=Floor
  Divide1 : Product  Inputs=*/
  Gain1 : Gain  Gain=2*pi
  IC : InitialCondition  Value=simIn.init.PIDA.TarFilt
  Logical Operator1 : Logic  Operator=OR  AllPortsSameDT=off  OutDataTypeStr=boolean
  Product : Product
  Product1 : Product
  Product2 : Product
  Subtract1 : Sum  Inputs=+-
  Sum : Sum  Inputs=++|
  Switch1 : Switch  Criteria=u2 > Threshold  SaturateOnIntegerOverflow=off  InputSameDT=off
  Unit Delay : UnitDelay  SampleTime=-1  HasFrameUpgradeWarning=on
  y : Outport
  wires:
  Product/1 -> Sum/1
  u/1 -> Product/2
  [alpha] -> Product/1
  Constant2/1 -> Subtract1/1
  [alpha] -> Subtract1/2
  Subtract1/1 -> Product1/1
  Product1/1 -> Sum/2
  Sum/1 -> IC/1
  Unit Delay/1 -> Product1/2
  IC/1 -> y/1, Unit Delay/1
  [cutoff_freq] -> Compare To Zero3/1
  Constant5/1 -> Product2/2
  Compare To Zero4/1 -> Product2/1
  Logical Operator1/1 -> Switch1/2
  Compare To Zero2/1 -> Logical Operator1/1
  cutoff_freq/1 -> [cutoff_freq]
  Switch1/1 -> [alpha]
  [cutoff_freq] -> Gain1/1
  Divide1/1 -> Add1/2
  [dt] -> Compare To Zero4/1
  Constant1/1 -> Divide1/1
  Data Type Conversion1/1 -> [dt]
  Product2/1 -> Switch1/1
  ATC input time constant1/1 -> Data Type Conversion1/1
  Compare To Zero3/1 -> Logical Operator1/2
  Gain1/1 -> Divide1/2
  [dt] -> Calculate Alpha1/1, Add1/1
  Add1/1 -> Calculate Alpha1/2
  Calculate Alpha1/1 -> Switch1/3
  [dt] -> Compare To Zero2/1

== system arducopter/Position Controller/PID Acceleration z/Slew Limiter ==
  note: Data Store Memory Elements: Global variables of subsystem
  note: Slew Limiter
      |
      | Calculates the slew limit modifiert Dmod for the P and D part of the controller. The calculation of Dmod is taken from SlewLimiter::modifier() in SlewLimiter.cpp.
  note: Alpha Calculation:
      | $\alpha = \frac{\mathrm{d}t}{\mathrm{d}t + 2 \pi f_{\mathrm{Cutoff}}$
  note: See AP_Math.cpp, calc_lowpass_alpha_dt()
  p_out : Inport
  sr_max : Inport  Port=2
  sr_tau : Inport  Port=3
  sr_flt_f : Inport  Port=4
  clock : Inport  Port=5
  d_out : Inport  Port=6
  ATC input time constant : Constant  Value=simIn.param.dt
  Add1 : Sum
  Calculate Alpha : Product  Inputs=*/
  Calculate Dmod : MATLAB Function  TreatAsAtomicUnit=on  SystemSampleTime=0.0025
  Compare To Zero2 : simulink/Logic and Bit Operations/Compare To Zero  relop=<=  OutDataTypeStr=boolean
  Compare To Zero3 : simulink/Logic and Bit Operations/Compare To Zero  relop=<=  OutDataTypeStr=boolean
  Compare To Zero4 : simulink/Logic and Bit Operations/Compare To Zero  relop=~=  OutDataTypeStr=boolean
  Constant1 : Constant  OutDataTypeStr=single
  Constant5 : Constant  OutDataTypeStr=single
  Data Store Memory : DataStoreMemory  DataStoreName=pos_event_stored  ReadBeforeWriteMsg=warning  WriteAfterWriteMsg=warning  WriteAfterReadMsg=warning  InitialValue=false  ShowAdditionalParam=off  OutDataTypeStr=boolean
  Data Store Memory1 : DataStoreMemory  DataStoreName=neg_event_stored  ReadBeforeWriteMsg=warning  WriteAfterWriteMsg=warning  WriteAfterReadMsg=warning  InitialValue=false  ShowAdditionalParam=off  OutDataTypeStr=boolean
  Data Store Memory10 : DataStoreMemory  DataStoreName=modifier_slew_rate  ReadBeforeWriteMsg=warning  WriteAfterWriteMsg=warning  WriteAfterReadMsg=warning  InitialValue=simIn.init.PIDA.SROut  ShowAdditionalParam=off  OutDataTypeStr=single
  Data Store Memory11 : DataStoreMemory  DataStoreName=output_slew_rate  ReadBeforeWriteMsg=warning  WriteAfterWriteMsg=warning  WriteAfterReadMsg=warning  InitialValue=simIn.init.PIDA.SROut  ShowAdditionalParam=off  OutDataTypeStr=single
  Data Store Memory2 : DataStoreMemory  DataStoreName=pos_event_idx  ReadBeforeWriteMsg=warning  WriteAfterWriteMsg=warning  WriteAfterReadMsg=warning  InitialValue=1  ShowAdditionalParam=off  OutDataTypeStr=int8
  Data Store Memory3 : DataStoreMemory  DataStoreName=neg_event_idx  ReadBeforeWriteMsg=warning  WriteAfterWriteMsg=warning  WriteAfterReadMsg=warning  InitialValue=1  ShowAdditionalParam=off  OutDataTypeStr=int8
  Data Store Memory4 : DataStoreMemory  DataStoreName=pos_event_ms  ReadBeforeWriteMsg=warning  WriteAfterWriteMsg=warning  WriteAfterReadMsg=warning  InitialValue=[0 0]  ShowAdditionalParam=off  OutDataTypeStr=uint32  Dimensions=2
  Data Store Memory5 : DataStoreMemory  DataStoreName=neg_event_ms  ReadBeforeWriteMsg=warning  WriteAfterWriteMsg=warning  WriteAfterReadMsg=warning  InitialValue=[0 0]  ShowAdditionalParam=off  OutDataTypeStr=uint32  Dimensions=2
  Data Store Memory6 : DataStoreMemory  DataStoreName=max_pos_slew_rate  ReadBeforeWriteMsg=warning  WriteAfterWriteMsg=warning  WriteAfterReadMsg=warning  ShowAdditionalParam=off  OutDataTypeStr=single
  Data Store Memory7 : DataStoreMemory  DataStoreName=max_pos_slew_event_ms  ReadBeforeWriteMsg=warning  WriteAfterWriteMsg=warning  WriteAfterReadMsg=warning  ShowAdditionalParam=off  OutDataTypeStr=uint32
  Data Store Memory8 : DataStoreMemory  DataStoreName=max_neg_slew_rate  ReadBeforeWriteMsg=warning  WriteAfterWriteMsg=warning  WriteAfterReadMsg=warning  ShowAdditionalParam=off  OutDataTypeStr=single
  Data Store Memory9 : DataStoreMemory  DataStoreName=max_neg_slew_event_ms  ReadBeforeWriteMsg=warning  WriteAfterWriteMsg=warning  WriteAfterReadMsg=warning  ShowAdditionalParam=off  OutDataTypeStr=uint32
  Data Store Read : DataStoreRead  DataStoreName=modifier_slew_rate  DataStoreElements=modifier_slew_rate  IndexOptions=Index vector (dialog)  Indices=1  OutputSizes=1
  Data Store Read1 : DataStoreRead  DataStoreName=output_slew_rate  DataStoreElements=output_slew_rate  IndexOptions=Index vector (dialog)  Indices=1  OutputSizes=1
  Data Type Conversion2 : DataTypeConversion  OutDataTypeStr=single  SaturateOnIntegerOverflow=off  RndMeth=Floor
  Divide1 : Product  Inputs=*/
  Gain1 : Gain  Gain=2*pi
  IC : InitialCondition  Value=2*simIn.init.PIDA.SROut
  Logical Operator1 : Logic  Operator=OR  AllPortsSameDT=off  OutDataTypeStr=boolean
  Lowpass Filter : MATLAB Function  TreatAsAtomicUnit=on
  Product2 : Product
  Subsystem : Subsystem
  Switch1 : Switch  Criteria=u2 > Threshold  SaturateOnIntegerOverflow=off  InputSameDT=off
  Terminator : Terminator
  Terminator1 : Terminator
  Unit Delay1 : UnitDelay  SampleTime=-1  HasFrameUpgradeWarning=on
  Dmod : Outport
  wires:
  Data Store Read/1 -> Terminator/1  "zAccSrMod"
  Data Store Read1/1 -> Terminator1/1  "zAccSrOut"
  Switch1/1 -> Lowpass Filter/2(alpha)
  sr_tau/1 -> Calculate Dmod/3(sr_tau)
  [dt] -> Calculate Alpha/1, Add1/1
  sr_flt_f/1 -> [cutoff_freq]
  Compare To Zero2/1 -> Logical Operator1/1
  Add1/1 -> Calculate Alpha/2
  Compare To Zero3/1 -> Logical Operator1/2
  Compare To Zero4/1 -> Product2/1
  Calculate Dmod/1(Dmod) -> Dmod/1  "zAccDmod"
  ATC input time constant/1 -> Data Type Conversion2/1
  [dt] -> Compare To Zero2/1
  Constant1/1 -> Divide1/1
  Data Type Conversion2/1 -> [dt]
  [dt] -> Calculate Dmod/4(dt)
  Unit Delay1/1 -> Lowpass Filter/3(out_last)
  Divide1/1 -> Add1/2
  Product2/1 -> Switch1/1
  Logical Operator1/1 -> Switch1/2
  [cutoff_freq] -> Gain1/1
  clock/1 -> Calculate Dmod/5(time)
  Constant5/1 -> Product2/2
  Lowpass Filter/1(out) -> IC/1  "zAccSrFilt"
  Calculate Alpha/1 -> Switch1/3
  IC/1 -> Calculate Dmod/1(slew_rate), Unit Delay1/1
  [dt] -> Compare To Zero4/1
  Gain1/1 -> Divide1/2
  sr_max/1 -> Calculate Dmod/2(sr_max)
  [cutoff_freq] -> Compare To Zero3/1
  Subsystem/1(sr_raw) -> Lowpass Filter/1(in)  "zAccSrRaw"
  p_out/1 -> Subsystem/1(p_out)
  d_out/1 -> Subsystem/2(d_out)

== system arducopter/Position Controller/PID Acceleration z/i_max check ==
  note: Ensure imax is always large enough to overpower hover throttle
      | Check for sufficient high imax is taken from AC_PosControl.cpp, line 984-986.
  thrHover : Inport
  i_max_ : Inport  Port=2
  Gain : Gain  Gain=1000
  Relational Operator : RelationalOperator  Operator=>  OutDataTypeStr=boolean  RndMeth=Simplest  InputSameDT=off
  Switch : Switch  Criteria=u2 > Threshold  SaturateOnIntegerOverflow=off  InputSameDT=off
  i_max : Outport
  wires:
  thrHover/1 -> Gain/1
  Gain/1 -> Switch/1, Relational Operator/1
  i_max_/1 -> Switch/3, Relational Operator/2
  Relational Operator/1 -> Switch/2
  Switch/1 -> i_max/1

== system arducopter/Position Controller/PID Velocity z/Calc Derivative ==
  e : Inport
  ATC input time constant : Constant  Value=simIn.param.dt
  Divide : Product  Inputs=*/
  Sum : Sum  Inputs=|+-
  Unit Delay : UnitDelay  SampleTime=-1  HasFrameUpgradeWarning=on
  derivative : Outport
  wires:
  e/1 -> Sum/1, Unit Delay/1
  Unit Delay/1 -> Sum/2
  Sum/1 -> Divide/1
  ATC input time constant/1 -> Divide/2
  Divide/1 -> derivative/1
